simulink model "LF_Week4_PD"  (R2025b)
settings: Solver=FixedStepDiscrete  StartTime=0.0  StopTime=cfg.stop_time  FixedStep=cfg.Ts  RelTol=1e-3
model workspace (MAT data in the model file):
  Kd = 0.03
  Kp = 0.45
  cfg.root = 'F:\DIGITAL TWEEN\line_follower_twin\weeks1_4'
  cfg.trackMask = [0 0 0 0 0 0 0 0 0 0 0 0 ... (276271 elements, 431x641)]
  cfg.trackReflectance = [0 0 0 0 0 0 0 0 0 0 0 0 ... (276271 elements, 431x641)]
  cfg.map_width_m = 2.56
  cfg.map_height_m = 1.72
  cfg.meters_per_pixel_x = 0.004
  cfg.meters_per_pixel_y = 0.004
  cfg.line_width_m = 0.02
  cfg.stroke_width_px = 5
  cfg.referenceXY = [0.48 0.484 0.488 0.492 0.496 0.5 0.504 0.508 0.512 0.516 0.52 0.524 ... (6258 elements, 3129x2)]
  cfg.referenceArc = [0 0.004 0.008 0.012 0.016 0.02 0.024 0.028 0.032 0.036 0.04 0.044 ... (3129 elements, 1x3129)]
  cfg.x0 = 0.48
  cfg.y0 = 0.196
  cfg.theta0 = 0
  cfg.Ts = 0.02
  cfg.wheel_base_m = 0.12
  cfg.body_length_m = 0.16
  cfg.body_width_m = 0.1
  cfg.sensor_front_m = 0.05
  cfg.sensor_spacing_m = 0.008
  cfg.sensor_weights = [3.5 2.5 1.5 0.5 -0.5 -1.5 -2.5 -3.5]
  cfg.km = 0.35
  cfg.base_speed = 0.35
  cfg.Kp = 0.45
  cfg.Kd = 0.03
  cfg.Ki = 0
  cfg.derivative_tau = 0.08
  cfg.sensor_threshold = 0.5
  cfg.loss_timeout_s = 0.2
  cfg.stop_time = 100
  cfg.results_dir = 'F:\DIGITAL TWEEN\line_follower_twin\weeks1_4\results'
  cfg.models_dir = 'F:\DIGITAL TWEEN\line_follower_twin\weeks1_4\models'
  uL = 0.5
  uR = 0.5
undefined symbols (not defined in the file): DiscIntNeverNeededParam
settings Model: Creator=Xiaol  LastModifiedBy=Xiaol
settings DataIOCC: SaveOutput=off  SignalLogging=off

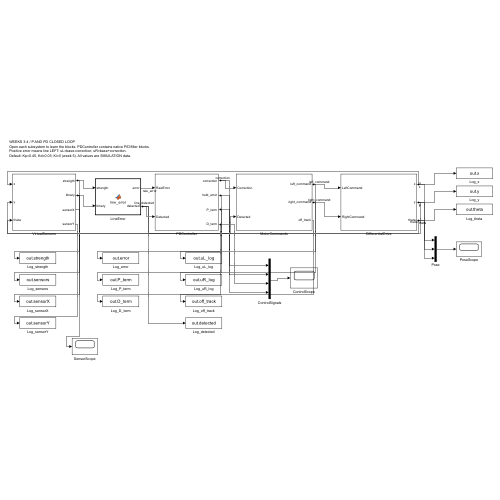
[thumbnail: Simulink's stored preview of the top-level diagram]
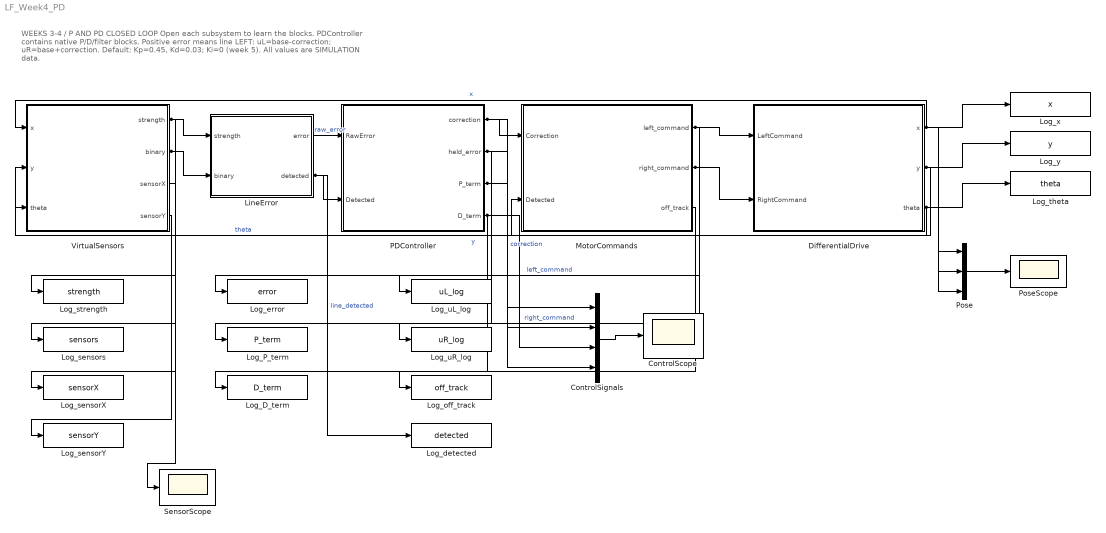
== system LF_Week4_PD ==
  note: WEEKS 3-4 / P AND PD CLOSED LOOP
      | Open each subsystem to learn the blocks. PDController contains native P/D/filter blocks.
      | Positive error means line LEFT: uL=base-correction; uR=base+correction.
      | Default: Kp=0.45, Kd=0.03; Ki=0 (week 5). All values are SIMULATION data.
  ControlScope : Scope
  ControlSignals : Mux
  DifferentialDrive : Subsystem
  LineError : MATLAB Function  TreatAsAtomicUnit=on
  Log_D_term : ToWorkspace  VariableName=D_term  SaveFormat=Timeseries  SampleTime=-1
  Log_P_term : ToWorkspace  VariableName=P_term  SaveFormat=Timeseries  SampleTime=-1
  Log_detected : ToWorkspace  VariableName=detected  SaveFormat=Timeseries  SampleTime=-1
  Log_error : ToWorkspace  VariableName=error  SaveFormat=Timeseries  SampleTime=-1
  Log_off_track : ToWorkspace  VariableName=off_track  SaveFormat=Timeseries  SampleTime=-1
  Log_sensorX : ToWorkspace  VariableName=sensorX  SaveFormat=Timeseries  SampleTime=-1
  Log_sensorY : ToWorkspace  VariableName=sensorY  SaveFormat=Timeseries  SampleTime=-1
  Log_sensors : ToWorkspace  VariableName=sensors  SaveFormat=Timeseries  SampleTime=-1
  Log_strength : ToWorkspace  VariableName=strength  SaveFormat=Timeseries  SampleTime=-1
  Log_theta : ToWorkspace  VariableName=theta  SaveFormat=Timeseries  SampleTime=-1
  Log_uL_log : ToWorkspace  VariableName=uL_log  SaveFormat=Timeseries  SampleTime=-1
  Log_uR_log : ToWorkspace  VariableName=uR_log  SaveFormat=Timeseries  SampleTime=-1
  Log_x : ToWorkspace  VariableName=x  SaveFormat=Timeseries  SampleTime=-1
  Log_y : ToWorkspace  VariableName=y  SaveFormat=Timeseries  SampleTime=-1
  MotorCommands : Subsystem
  PDController : Subsystem
  Pose : Mux  Inputs=3
  PoseScope : Scope
  SensorScope : Scope
  VirtualSensors : Subsystem
  wires:
  DifferentialDrive/1(x) -> Log_x/1, Pose/1, VirtualSensors/1(x)  "x"
  DifferentialDrive/2(y) -> Log_y/1, Pose/2, VirtualSensors/2(y)  "y"
  DifferentialDrive/3(theta) -> Log_theta/1, Pose/3, VirtualSensors/3(theta)  "theta"
  Pose/1 -> PoseScope/1
  VirtualSensors/1(strength) -> LineError/1(strength), Log_strength/1
  VirtualSensors/2(binary) -> LineError/2(binary), Log_sensors/1, SensorScope/1
  LineError/1(error) -> PDController/1(RawError)  "raw_error"
  LineError/2(detected) -> PDController/2(Detected), MotorCommands/2(Detected), Log_detected/1  "line_detected"
  PDController/1(correction) -> MotorCommands/1(Correction), ControlSignals/4  "correction"
  MotorCommands/1(left_command) -> DifferentialDrive/1(LeftCommand), Log_uL_log/1  "left_command"
  MotorCommands/2(right_command) -> DifferentialDrive/2(RightCommand), Log_uR_log/1  "right_command"
  VirtualSensors/3(sensorX) -> Log_sensorX/1
  VirtualSensors/4(sensorY) -> Log_sensorY/1
  PDController/2(held_error) -> Log_error/1, ControlSignals/1
  PDController/3(P_term) -> Log_P_term/1, ControlSignals/2
  PDController/4(D_term) -> Log_D_term/1, ControlSignals/3
  MotorCommands/3(off_track) -> Log_off_track/1
  ControlSignals/1 -> ControlScope/1

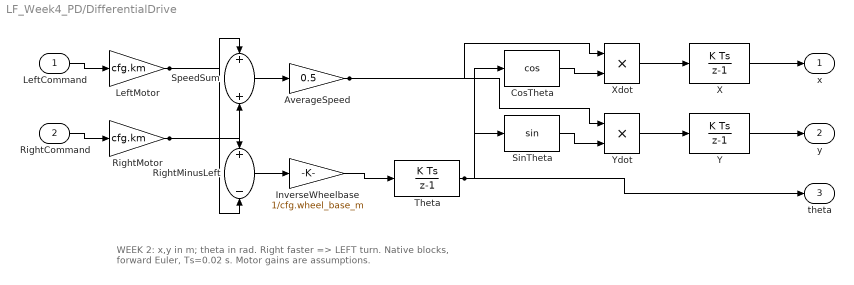
== system LF_Week4_PD/DifferentialDrive ==
  note: WEEK 2: x,y in m; theta in rad. Right faster => LEFT turn.
      | Native blocks, forward Euler, Ts=0.02 s. Motor gains are assumptions.
  LeftCommand : Inport
  RightCommand : Inport  Port=2
  AverageSpeed : Gain  Gain=0.5
  CosTheta : Trigonometry  Operator=cos
  InverseWheelbase : Gain  Gain=1/cfg.wheel_base_m
  LeftMotor : Gain  Gain=cfg.km
  RightMinusLeft : Sum  Inputs=+-
  RightMotor : Gain  Gain=cfg.km
  SinTheta : Trigonometry
  SpeedSum : Sum
  Theta : DiscreteIntegrator  gainval=1  InitialCondition=cfg.theta0  SampleTime=cfg.Ts  ICPrevOutput=DiscIntNeverNeededParam  ICPrevScaledInput=DiscIntNeverNeededParam
  X : DiscreteIntegrator  gainval=1  InitialCondition=cfg.x0  SampleTime=cfg.Ts  ICPrevOutput=DiscIntNeverNeededParam  ICPrevScaledInput=DiscIntNeverNeededParam
  Xdot : Product
  Y : DiscreteIntegrator  gainval=1  InitialCondition=cfg.y0  SampleTime=cfg.Ts  ICPrevOutput=DiscIntNeverNeededParam  ICPrevScaledInput=DiscIntNeverNeededParam
  Ydot : Product
  x : Outport
  y : Outport  Port=2
  theta : Outport  Port=3
  wires:
  LeftCommand/1 -> LeftMotor/1
  RightCommand/1 -> RightMotor/1
  LeftMotor/1 -> SpeedSum/1, RightMinusLeft/2
  RightMotor/1 -> SpeedSum/2, RightMinusLeft/1
  SpeedSum/1 -> AverageSpeed/1
  RightMinusLeft/1 -> InverseWheelbase/1
  InverseWheelbase/1 -> Theta/1
  Theta/1 -> CosTheta/1, SinTheta/1, theta/1
  AverageSpeed/1 -> Xdot/1, Ydot/1
  CosTheta/1 -> Xdot/2
  SinTheta/1 -> Ydot/2
  Xdot/1 -> X/1
  Ydot/1 -> Y/1
  X/1 -> x/1
  Y/1 -> y/1

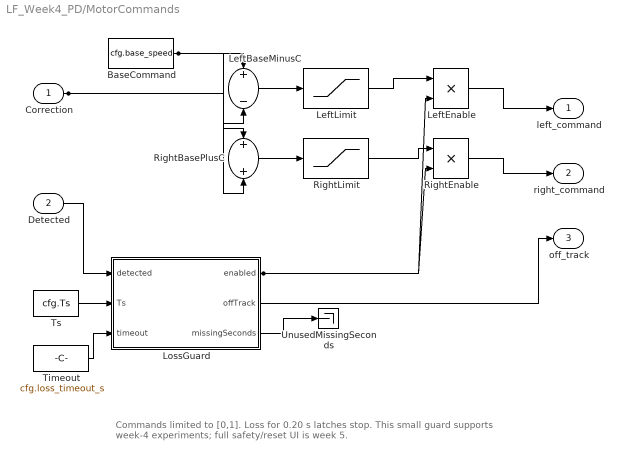
== system LF_Week4_PD/MotorCommands ==
  note: Commands limited to [0,1]. Loss for 0.20 s latches stop.
      | This small guard supports week-4 experiments; full safety/reset UI is week 5.
  Correction : Inport
  Detected : Inport  Port=2
  BaseCommand : Constant  Value=cfg.base_speed  SampleTime=cfg.Ts
  LeftBaseMinusC : Sum  Inputs=+-
  LeftEnable : Product
  LeftLimit : Saturate  UpperLimit=1  LowerLimit=0
  LossGuard : MATLAB Function  TreatAsAtomicUnit=on
  RightBasePlusC : Sum
  RightEnable : Product
  RightLimit : Saturate  UpperLimit=1  LowerLimit=0
  Timeout : Constant  Value=cfg.loss_timeout_s
  Ts : Constant  Value=cfg.Ts
  UnusedMissingSeconds : Terminator
  left_command : Outport
  right_command : Outport  Port=2
  off_track : Outport  Port=3
  wires:
  Detected/1 -> LossGuard/1(detected)
  Ts/1 -> LossGuard/2(Ts)
  Timeout/1 -> LossGuard/3(timeout)
  BaseCommand/1 -> LeftBaseMinusC/1, RightBasePlusC/1
  Correction/1 -> LeftBaseMinusC/2, RightBasePlusC/2
  LeftBaseMinusC/1 -> LeftLimit/1
  RightBasePlusC/1 -> RightLimit/1
  LeftLimit/1 -> LeftEnable/1
  LossGuard/1(enabled) -> LeftEnable/2, RightEnable/2
  RightLimit/1 -> RightEnable/1
  LeftEnable/1 -> left_command/1
  RightEnable/1 -> right_command/1
  LossGuard/2(offTrack) -> off_track/1
  LossGuard/3(missingSeconds) -> UnusedMissingSeconds/1

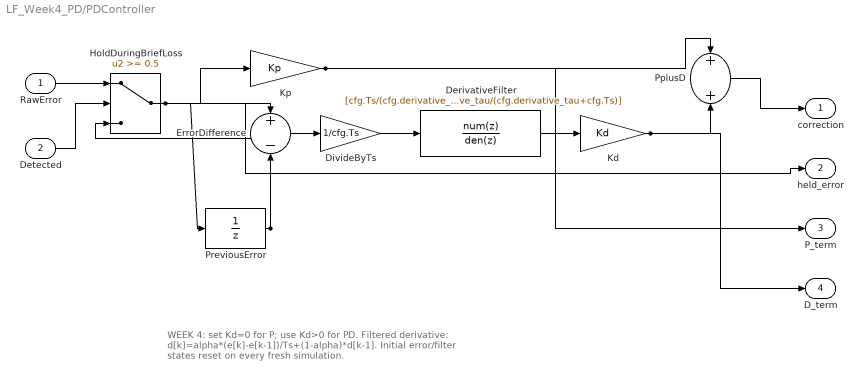
== system LF_Week4_PD/PDController ==
  note: WEEK 4: set Kd=0 for P; use Kd>0 for PD.
      | Filtered derivative: d[k]=alpha*(e[k]-e[k-1])/Ts+(1-alpha)*d[k-1].
      | Initial error/filter states reset on every fresh simulation.
  RawError : Inport
  Detected : Inport  Port=2
  DerivativeFilter : DiscreteTransferFcn  Numerator=[cfg.Ts/(cfg.derivative_tau+cfg.Ts) 0]  Denominator=[1 -cfg.derivative_tau/(cfg.derivative_tau+cfg.Ts)]  SampleTime=cfg.Ts
  DivideByTs : Gain  Gain=1/cfg.Ts
  ErrorDifference : Sum  Inputs=+-
  HoldDuringBriefLoss : Switch  Threshold=0.5  SaturateOnIntegerOverflow=off  InputSameDT=off
  Kd : Gain  Gain=Kd
  Kp : Gain  Gain=Kp
  PplusD : Sum
  PreviousError : UnitDelay  SampleTime=cfg.Ts  HasFrameUpgradeWarning=on
  correction : Outport
  held_error : Outport  Port=2
  P_term : Outport  Port=3
  D_term : Outport  Port=4
  wires:
  RawError/1 -> HoldDuringBriefLoss/1
  Detected/1 -> HoldDuringBriefLoss/2
  PreviousError/1 -> HoldDuringBriefLoss/3, ErrorDifference/2
  HoldDuringBriefLoss/1 -> PreviousError/1, Kp/1, ErrorDifference/1, held_error/1
  ErrorDifference/1 -> DivideByTs/1
  DivideByTs/1 -> DerivativeFilter/1
  DerivativeFilter/1 -> Kd/1
  Kp/1 -> PplusD/1, P_term/1
  Kd/1 -> PplusD/2, D_term/1
  PplusD/1 -> correction/1

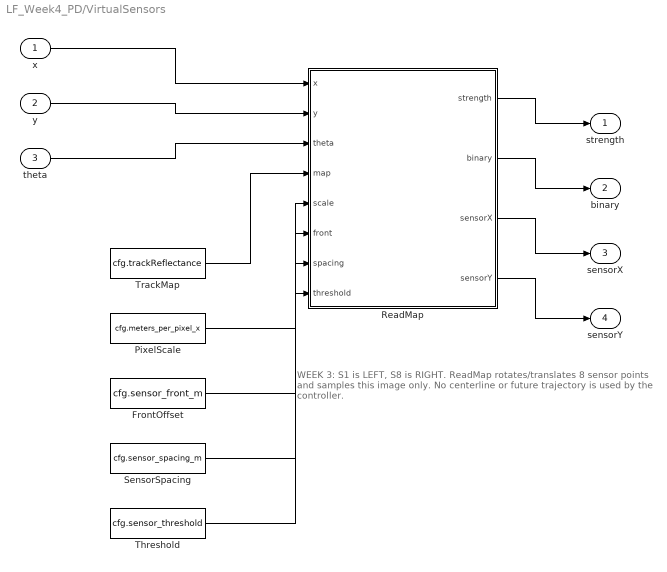
== system LF_Week4_PD/VirtualSensors ==
  note: WEEK 3: S1 is LEFT, S8 is RIGHT.
      | ReadMap rotates/translates 8 sensor points and samples this image only.
      | No centerline or future trajectory is used by the controller.
  x : Inport
  y : Inport  Port=2
  theta : Inport  Port=3
  FrontOffset : Constant  Value=cfg.sensor_front_m
  PixelScale : Constant  Value=cfg.meters_per_pixel_x
  ReadMap : MATLAB Function  TreatAsAtomicUnit=on
  SensorSpacing : Constant  Value=cfg.sensor_spacing_m
  Threshold : Constant  Value=cfg.sensor_threshold
  TrackMap : Constant  Value=cfg.trackReflectance
  strength : Outport
  binary : Outport  Port=2
  sensorX : Outport  Port=3
  sensorY : Outport  Port=4
  wires:
  x/1 -> ReadMap/1(x)
  y/1 -> ReadMap/2(y)
  theta/1 -> ReadMap/3(theta)
  TrackMap/1 -> ReadMap/4(map)
  PixelScale/1 -> ReadMap/5(scale)
  FrontOffset/1 -> ReadMap/6(front)
  SensorSpacing/1 -> ReadMap/7(spacing)
  Threshold/1 -> ReadMap/8(threshold)
  ReadMap/1(strength) -> strength/1
  ReadMap/2(binary) -> binary/1
  ReadMap/3(sensorX) -> sensorX/1
  ReadMap/4(sensorY) -> sensorY/1

== matlab function LF_Week4_PD/LineError ==
  data: strength input; error output; binary input; detected output
function [error,detected] = line_error(strength,binary)
%#codegen
% Positive error: black line is on the LEFT, so increase right-side speed.
detected=double(any(binary>0.5));
error=0;
if detected
    total=0; weighted=0;
    for i=1:8
        total=total+strength(i);
        weighted=weighted+strength(i)*(4.5-i);
    end
    error=weighted/(3.5*max(total,1e-12));
end
end

== matlab function LF_Week4_PD/VirtualSensors/ReadMap ==
  data: x input; strength output; y input; theta input; map input; scale input; front input; spacing input; threshold input; binary output; sensorX output; sensorY output
function [strength,binary,sensorX,sensorY] = virtual_sensors(x,y,theta,map,scale,front,spacing,threshold)
%#codegen
% S1..S8 run LEFT to RIGHT as seen looking forward. Outside-map values are zero.
strength=zeros(1,8); binary=zeros(1,8);
sensorX=zeros(1,8); sensorY=zeros(1,8);
[H,W]=size(map);
ct=cos(theta); st=sin(theta);
for i=1:8
    localY=(4.5-i)*spacing;
    X=x+ct*front-st*localY;
    Y=y+st*front+ct*localY;
    sensorX(i)=X; sensorY(i)=Y;
    col=1+X/scale; row=H-Y/scale;
    if col>=1 && col<=W && row>=1 && row<=H
        c0=floor(col); r0=floor(row);
        c1=min(c0+1,W); r1=min(r0+1,H);
        dc=col-c0; dr=row-r0;
        strength(i)=(1-dr)*((1-dc)*map(r0,c0)+dc*map(r0,c1)) ...
                   +dr*((1-dc)*map(r1,c0)+dc*map(r1,c1));
    end
    binary(i)=double(strength(i)>=threshold);
end
end

== matlab function LF_Week4_PD/MotorCommands/LossGuard ==
  data: detected input; enabled output; Ts input; timeout input; offTrack output; missingSeconds output
function [enabled,offTrack,missingSeconds] = loss_guard(detected,Ts,timeout)
%#codegen
% Minimal protection: after continuous loss, latch STOP until a fresh run/reset.
persistent elapsed active stopped
if isempty(elapsed),elapsed=0;active=false;stopped=false;end
if detected
    elapsed=0;active=false;
elseif active
    elapsed=elapsed+Ts;
else
    elapsed=0;active=true; % the first missing sample marks the start of loss
end
if elapsed>=timeout-1e-12,stopped=true;end
enabled=double(~stopped);
offTrack=double(stopped);
missingSeconds=elapsed;
end
